simulink model "buck_converter_NM"  (R2017b)
settings: Solver=VariableStepAuto  StartTime=0.0  StopTime=5  RelTol=1e-3
libraries: powerlib x8
settings Model: Creator=priya  LastModifiedBy=VIJAYPRASATH
settings DataIOCC: ReturnWorkspaceOutputs=on
settings DebuggingCC: UnconnectedInputMsg=none  UnconnectedOutputMsg=none  UnconnectedLineMsg=none
settings ModelReferenceCC: EnableRefExpFcnMdlSchedulingChecks=off
settings SFSimCC: SimUseLocalCustomCode=on
settings RTWCC: Description=Generic Real-Time Target  RTWUseLocalCustomCode=on

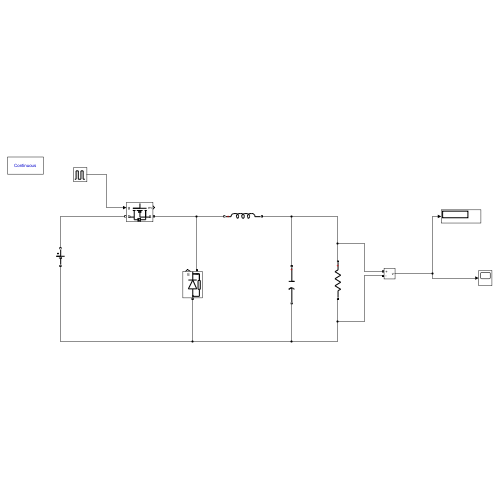
[thumbnail: Simulink's stored preview of the top-level diagram]
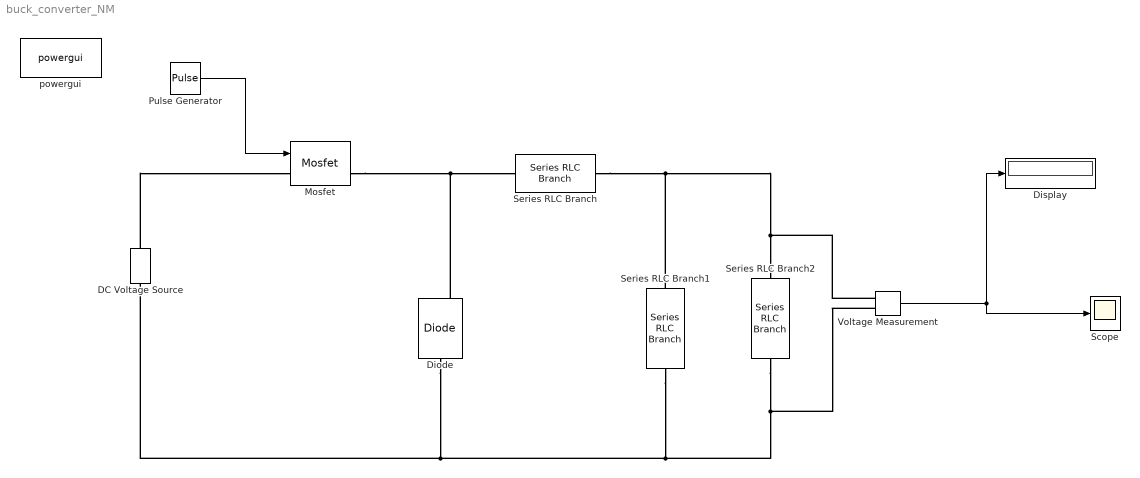
== system buck_converter_NM ==
  DC Voltage Source : powerlib/Electrical Sources/DC Voltage Source  Amplitude=48  Measurements=Voltage
  Diode : powerlib/Power Electronics/Diode  Ron=0.001  Lon=0  Vf=0.8  IC=0  UseSnubber=0  Rs=500  Cs=250e-9  Measurements=on
  Display : Display
  Mosfet : powerlib/Power Electronics/Mosfet  Ron=0.1  Lon=0  Rd=0.01  Vfd=0.7  IC=0  Rs=1e5  Cs=inf  Measurements=on
  Pulse Generator : DiscretePulseGenerator  PulseType=Time based  Period=2.5e-5  PulseWidth=31.25
  Scope : Scope
  Series RLC Branch : powerlib/Elements/Series RLC Branch  LConnTagsString=__new0  RConnTagsString=__new0  BranchType=L  Resistance=1  Inductance=85.93e-6  SetiL0=off  InitialCurrent=0  Capacitance=1e-6  Setx0=off  InitialVoltage=0  Measurements=None
  Series RLC Branch1 : powerlib/Elements/Series RLC Branch  LConnTagsString=__new0  RConnTagsString=__new0  BranchType=C  Resistance=1  Inductance=1e-3  SetiL0=off  InitialCurrent=0  Capacitance=12.5e-6  Setx0=off  InitialVoltage=0  Measurements=None
  Series RLC Branch2 : powerlib/Elements/Series RLC Branch  LConnTagsString=__new0  RConnTagsString=__new0  BranchType=R  Resistance=8  Inductance=1e-3  SetiL0=off  InitialCurrent=0  Capacitance=1e-6  Setx0=off  InitialVoltage=0  Measurements=None
  Voltage Measurement : powerlib/Measurements/Voltage Measurement  PhasorSimulation=off  OutputType=Complex  PSBequivalent=0
  powergui : powerlib/powergui  Priority=1  SimulationMode=Continuous  SampleTime=50e-6  frequency=60  Iterations=50  frequencyindice=0  Pbase=100e6  ErrMax=1e-4  UnitsV=kV  UnitsW=MW  buscounter=0  FunctionMessages=off  echomessages=off  EnableUseOfTLC=off  CurrentSourceSwitches=off  DisableSnubberDevices=off  DisableRonSwitches=off  DisableVfSwitches=off  DisplayEquations=off  AutomaticDiscreteSolvers=off  SolverType=Tustin/Backward Euler (TBE)  Interpol=off  ExternalGateDelay=off  methode=off  Ts=100  x0status=blocks  SPID=on  SwTol=0  HookPort=off  NonlinearTolerance=1e-4  nMaxIteration=100  ContinueOnMaxIteration=off  RestoreLinks=warning  ResistiveCurrentMeasurement=off  Frange=[0:2:500]  Ylog=off  Xlog=on  ShowGrid=off  save=off  variable=ZData  structure=0  ZoomFFT=off  StartTime=0.0  cycles=1  DisplayStyle=1  fundamental=60  FreqAxis=off  MaxFrequency=1000  frequencyindicesteady=1  RmsSteady=1  display=off
  wires:
  Voltage Measurement/1 -> Display/1, Scope/1
  Pulse Generator/1 -> Mosfet/1
  connections:
  DC Voltage Source/RConn1 -- Mosfet/LConn1
  Mosfet/RConn1 -- Diode/RConn1 -- Series RLC Branch/LConn1
  Series RLC Branch/RConn1 -- Series RLC Branch1/LConn1 -- Voltage Measurement/LConn1 -- Series RLC Branch2/LConn1
  Series RLC Branch2/RConn1 -- Voltage Measurement/LConn2 -- Series RLC Branch1/RConn1 -- Diode/LConn1 -- DC Voltage Source/LConn1
